simulink model "RLSS_Physical"  (R2024b)
settings: Solver=ode45  StartTime=0.0  StopTime=5.0  RelTol=1e-5  AbsTol=1e-7
settings Model: Creator=Sadia Dina  LastModifiedBy=Sadia Dina

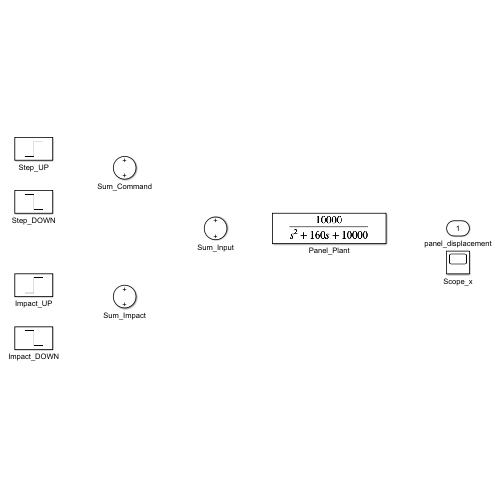
[thumbnail: Simulink's stored preview of the top-level diagram]
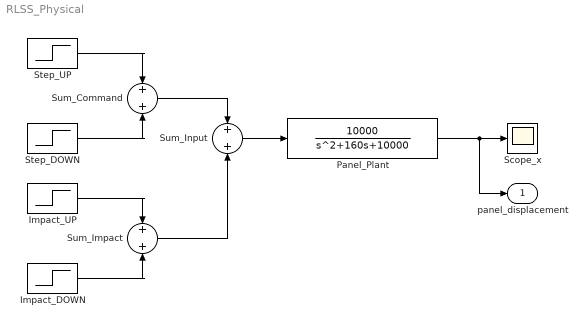
== system RLSS_Physical ==
  Impact_DOWN : Step  Time=1.5  After=-0.001  SampleTime=0
  Impact_UP : Step  Time=1.0  After=0.001  SampleTime=0
  Panel_Plant : TransferFcn  Numerator=[10000]  Denominator="[1  160  10000]"
  Scope_x : Scope
  Step_DOWN : Step  Time=2.5  After=-0.01  SampleTime=0
  Step_UP : Step  Time=0.5  After=0.01  SampleTime=0
  Sum_Command : Sum
  Sum_Impact : Sum
  Sum_Input : Sum
  panel_displacement : Outport
  wires:
  Panel_Plant/1 -> panel_displacement/1, Scope_x/1
  Sum_Input/1 -> Panel_Plant/1
  Sum_Impact/1 -> Sum_Input/2
  Impact_DOWN/1 -> Sum_Impact/2
  Impact_UP/1 -> Sum_Impact/1
  Step_DOWN/1 -> Sum_Command/2
  Step_UP/1 -> Sum_Command/1
  Sum_Command/1 -> Sum_Input/1
